simulink model "ADRC_PTAR2"  (R2025b)
settings: Solver=VariableStepAuto  StartTime=0.0  StopTime=500000  RelTol=1e-3
undefined symbols (not defined in the file): a0, a1, a2, a3, a4, a5, A_o, b0, Bau, denC, denGpi, E1, K, k, L, L_E, m, numC, numGpi, P_, Tau, Y_A, Y_H
libraries: slpidlib x1
settings Model: Creator=esteban  LastModifiedBy=esteban

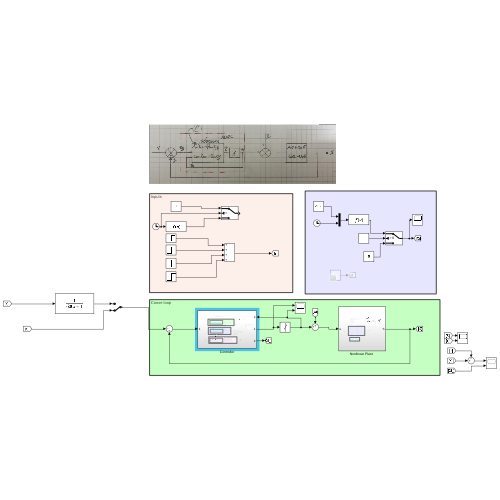
[thumbnail: Simulink's stored preview of the top-level diagram]
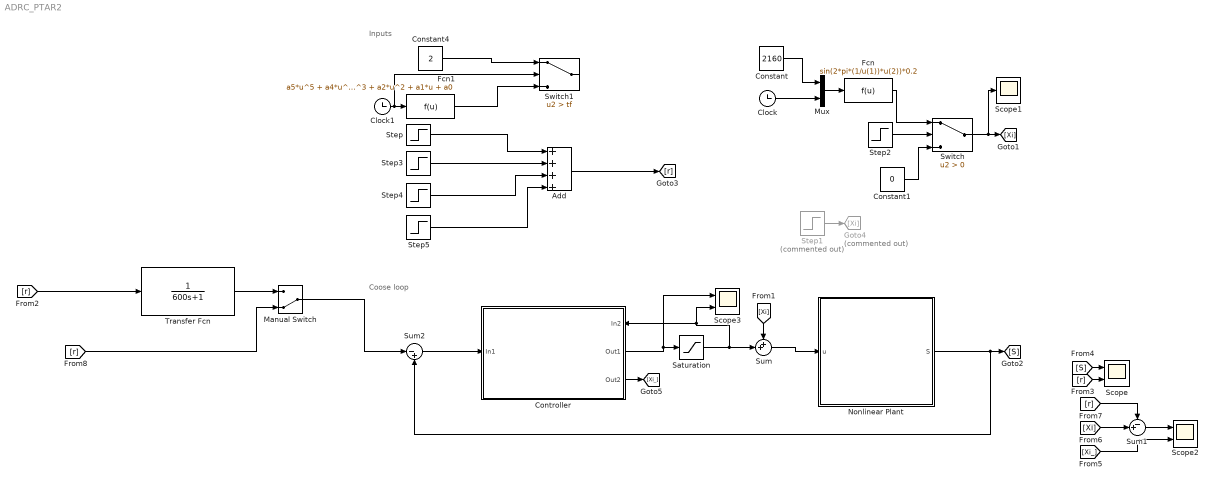
== system ADRC_PTAR2 ==
  note: Inputs
  note: Coose loop
  Add : Sum  Inputs=++++
  Clock : Clock
  Clock1 : Clock
  Constant : Constant  Value=2160
  Constant1 : Constant  Value=0
  Constant4 : Constant  Value=2
  Controller : Subsystem
      settings: PortSchema="{\"entries\":[{\"content\":{\"sides\":[{\"content\":{\"connectorIds\":[\"In1\"]},\"type\":\"ConnectorPlacement.EquallySpacedRectSide\",\"uuid\":\"f8461a81-2045-427e-a01f-edb502a076ed\"},{\"content\":{\"connectorIds\":[\"In2\",\"Out1\",\"Out2\"],\"side\":\"RIGHT\"},\"type\":\"ConnectorPlacement.EquallySpacedRectSide\",\"uuid\":\"3759dbef-32e7-4c7e-81ac-95d511493371\"},{\"content\":{\"side\":\"TOP\"},\"type\":\"ConnectorPlacement.EquallySpacedRectSide\",\"uuid\":\"15238c06-ddee-41c5-98cd-ddd7661e75a4\"}]},\"type\":\"ConnectorPlacement.EquallySpacedConnector\",\"uuid\":\"b42b1071-4ba9-4a20-bc2c-50f933ed0d4a\"}],\"packageUris\":[\"http://schema.mathworks.com/mf0/Connector/R2020b\"],\"version\":\"1.0\"}"
  Fcn : Fcn  Expr=sin(2*pi*(1/u(1))*u(2))*0.2
  Fcn1 : Fcn  Expr=a5*u^5 + a4*u^4 + a3*u^3 + a2*u^2 + a1*u + a0
  Goto4 : Goto  Commented=on  GotoTag=Xi
  Manual Switch : ManualSwitch  CurrentSetting=0
  Mux : Mux  Inputs=2
  "Nonlinear Plant  " : Subsystem
  Saturation : Saturate  UpperLimit=100  LowerLimit=0
  Scope : Scope  NumInputPorts=2
      settings: ActiveDisplayYMinimum=0.10311657808400376  ActiveDisplayYMaximum=3.8920516951737838
  Scope1 : Scope
      settings: ActiveDisplayYMinimum=-0.024830958943548569  ActiveDisplayYMaximum=0.2234786304919372  DataLoggingVariableName=ScopeData2
  Scope2 : Scope  NumInputPorts=2
      settings: ActiveDisplayYMinimum=-2.2923205992555511  ActiveDisplayYMaximum=4.2391627723615954  DataLoggingVariableName=ScopeData3
  Scope3 : Scope  NumInputPorts=2
      settings: ActiveDisplayYMinimum=-13.796251760586394  ActiveDisplayYMaximum=71.9907618847564  DataLoggingVariableName=ScopeData4
  Step : Step  Time=40000  After=2  SampleTime=0
  Step1 : Step  Commented=on  Time=4000  After=0.1  SampleTime=0
  Step2 : Step  Time=4000  SampleTime=0
  Step3 : Step  Time=80000  After=0.4  SampleTime=0
  Step4 : Step  Time=120000  After=-0.9  SampleTime=0
  Step5 : Step  Time=160000  After=0.5  SampleTime=0
  Sum : Sum  Inputs=++|
  Sum1 : Sum  Inputs=-+|
  Sum2 : Sum  Inputs=|-+
  Switch : Switch  Criteria=u2 > Threshold  SaturateOnIntegerOverflow=off  InputSameDT=off
  Switch1 : Switch  Criteria=u2 > Threshold  Threshold=tf  SaturateOnIntegerOverflow=off  InputSameDT=off
  Transfer Fcn : TransferFcn  Denominator=[600 1]
  wires:
  Mux/1 -> Fcn/1
  Clock/1 -> Mux/2
  Constant/1 -> Mux/1
  Step1/1 -> Goto4/1
  "Nonlinear Plant  "/1(S) -> [S], Sum2/2
  Constant1/1 -> Switch/3
  Fcn/1 -> Switch/1
  Step2/1 -> Switch/2
  Switch/1 -> Scope1/1, [Xi]
  [r] -> Scope/2
  Controller/2(Out2) -> [Xi_]
  [S] -> Scope/1
  [Xi_] -> Scope2/2
  Sum1/1 -> Scope2/1
  [r] -> Sum1/1
  Step/1 -> Add/1
  Step3/1 -> Add/2
  Step4/1 -> Add/3
  Step5/1 -> Add/4
  [Xi] -> Sum1/2
  Sum2/1 -> Controller/1(In1)
  [r] -> Transfer Fcn/1
  Manual Switch/1 -> Sum2/1
  Transfer Fcn/1 -> Manual Switch/1
  Sum/1 -> "Nonlinear Plant  "/1(u)
  Controller/1(Out1) -> Saturation/1, Scope3/1
  [r] -> Manual Switch/2
  Constant4/1 -> Switch1/1
  Clock1/1 -> Switch1/2, Fcn1/1
  Fcn1/1 -> Switch1/3
  Add/1 -> [r]
  Saturation/1 -> Scope3/2, Controller/2(In2), Sum/2
  [Xi] -> Sum/1

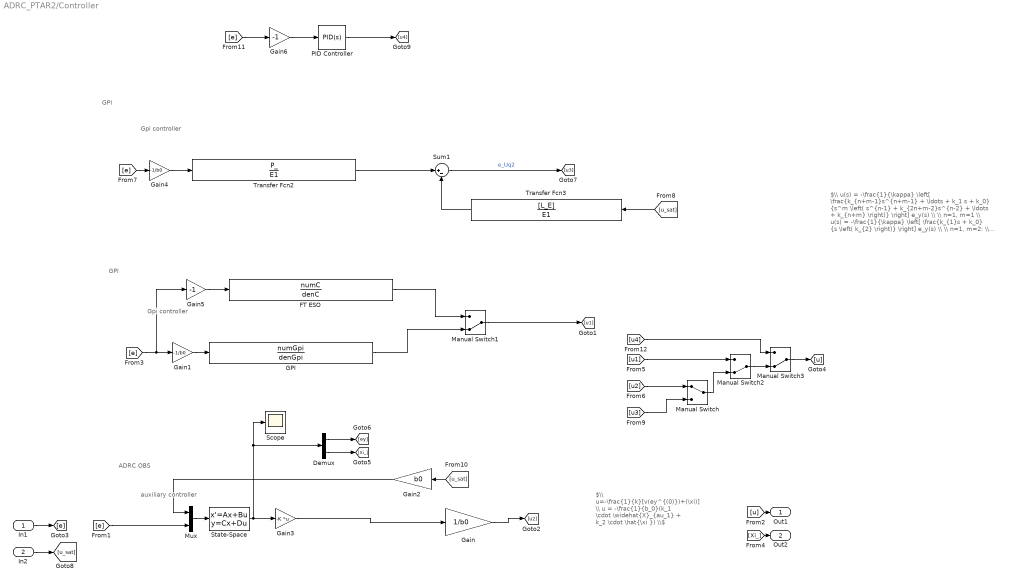
== system ADRC_PTAR2/Controller ==
  note: $\\ u(s) = -\frac{1}{\kappa} \left[ \frac{k_{n+m-1}s^{n+m-1} + \ldots + k_1 s + k_0} {s^m \left( s^{n-1} + k_{2n+m-2}s^{n-2} + \ldots + k_{n+m} \right)} \right] e_y(s) \\ \\ n=1, m=1 \\ u(s) = -\frac{1}{\kappa} \left[ \frac{k_{1}s + k_0} {s \left( k_{2} \right)} \right] e_y(s) \\ \\ n=1, m=2: \\ u(s) = -\frac{1}{b_0} \left[ \frac{k_{2}s^2+k_{1}s + k_0} {s^2} \right] e_y(s)$
  note: $\\ u=-\frac{1}{k}[v(ey^{(0)})+(\xi)] \\ u = -\frac{1}{b_0}(k_1 \cdot \widehat{X}_{au_1} + k_2 \cdot \hat{\xi }) \\$
  note: auxiliary controller
  note: Gpi controller
  note: GPI
  note: ADRC OBS
  note: GPI
  note: Gpi controller
  In1 : Inport
  In2 : Inport  Port=2
  Demux : Demux  Outputs=2
  FT ESO : TransferFcn  Numerator=numC  Denominator=denC
  GPI : TransferFcn  Numerator=numGpi  Denominator=denGpi
  Gain : Gain  Gain=1/b0
  Gain1 : Gain  Gain=-1/b0
  Gain2 : Gain  Gain=b0
  Gain3 : Gain  Gain=-K  Multiplication=Matrix(K*u)
  Gain4 : Gain  Gain=-1/b0
  Gain5 : Gain  Gain=-1
  Gain6 : Gain  Gain=-1
  Manual Switch : ManualSwitch
  Manual Switch1 : ManualSwitch  CurrentSetting=0
  Manual Switch2 : ManualSwitch  CurrentSetting=0
  Manual Switch3 : ManualSwitch  CurrentSetting=0
  Mux : Mux  Inputs=2
  PID Controller : slpidlib/PID Controller  Controller=PID  Form=Ideal  TimeDomain=Continuous-time  UseExternalTs=off  SampleTime=-1  IntegratorMethod=Forward Euler  FilterMethod=Forward Euler  ControllerParametersSource=internal  P=490.3  I=1/134.1  UseKiTs=off  D=14.78  UseExternalDerivativeSource=off  N=1/1.48  UseFilter=on  TunerSelectOption=Transfer Function Based (PID Tuner App)  InitialConditionSource=internal  InitialConditionForIntegrator=0  InitialConditionForFilter=0  DifferentiatorICPrevScaledInput=0  ExternalReset=none  TrackingMode=off  Kt=1  LimitOutput=off  SatLimitsSource=internal  UpperSaturationLimit=inf  LowerSaturationLimit=-inf  LinearizeAsGain=on  AntiWindupMode=none  Kb=1  LimitIntegrator=off  UpperIntegratorSaturationLimit=inf  LowerIntegratorSaturationLimit=-inf  POutMin=[]  POutMax=[]  IOutMin=[]  IOutMax=[]  DOutMin=[]  DOutMax=[]  NOutMin=[]  NOutMax=[]  SumOutMin=[]  SumOutMax=[]  SaturationOutMin=[]  SaturationOutMax=[]  PParamMin=[]  PParamMax=[]  IParamMin=[]  IParamMax=[]  DParamMin=[]  DParamMax=[]  NParamMin=[]  NParamMax=[]  KbParamMin=[]  KbParamMax=[]  KtParamMin=[]  KtParamMax=[]  KbOutMin=[]  KbOutMax=[]  KtOutMin=[]  KtOutMax=[]  IntegratorOutMin=[]  IntegratorOutMax=[]  FilterOutMin=[]  FilterOutMax=[]  SumI1OutMin=[]  SumI1OutMax=[]  SumI2OutMin=[]  SumI2OutMax=[]  SumI3OutMin=[]  SumI3OutMax=[]  SumI4OutMin=[]  SumI4OutMax=[]  SumDOutMin=[]  SumDOutMax=[]  DifferentiatorOutMin=[]  DifferentiatorOutMax=[]  FilterDiffOutCoefMin=[]  FilterDiffOutCoefMax=[]  ReciprocalOutMin=[]  ReciprocalOutMax=[]  SumDenOutMin=[]  SumDenOutMax=[]  SumNumOutMin=[]  SumNumOutMax=[]  DivideOutMin=[]  DivideOutMax=[]  UdiffTsProdOutMin=[]  UdiffTsProdOutMax=[]  NTsProdOutMin=[]  NTsProdOutMax=[]  UintegralTsProdOutMin=[]  UintegralTsProdOutMax=[]  UngainTsProdOutMin=[]  UngainTsProdOutMax=[]  ClampingZeroOutDataTypeStr=Inherit: Inherit via back propagation  ClampingZeroOutMin=[]  ClampingZeroOutMax=[]  FilterDenConstantOutDataTypeStr=Inherit: Inherit via back propagation  FilterDenConstantOutMin=[]  FilterDenConstantOutMax=[]  PCopyOutDataTypeStr=Inherit: Inherit via back propagation  PCopyOutMin=[]  PCopyOutMax=[]  NCopyOutDataTypeStr=Inherit: Inherit via back propagation  NCopyOutMin=[]  NCopyOutMax=[]  IntegratorContinuousStateAttributes=''  IntegratorStateMustResolveToSignalObject=off  IntegratorRTWStateStorageClass=Auto  FilterContinuousStateAttributes=''  FilterStateMustResolveToSignalObject=off  FilterRTWStateStorageClass=Auto  ParallelPVariant=Passthrough  IdealPVariant=InternalParameters  IVariant=InternalParameters  DVariant=InternalParameters  IntegratorVariant=Continuous  SatVariant=Disabled  AWVariant=Passthrough  PCopyVariant=Disabled  TRVariant=Disabled  FdbkBlocksVariant=Forward  IdealPFdbkVariant=Disabled  SatFdbkVariant=Disabled  DerivativeFilterVariant=ContFilter  NVariant=InternalParameters  NCopyVariant=Disabled  FilterICVariant=InternalICsFilter  IntegratorICVariant=InternalICs  ExternalResetVariant=Disabled  TRSumVariant=Passthrough  SumFdbkVariant=Disabled  SumVariant=Sum_PID  TsampFilterVariant=InternalTs  TsampNgainVariant=Passthrough  TsampIntegralVariant=Disabled_SignalSpec  ExternalSaturationOutDataTypeStr=Inherit: Same as second input  DerivativeSourceVariant=ErrorSignal  PreIntVariant=InternalPreInt
  Scope : Scope
      settings: ActiveDisplayYMinimum=-0.028041843832660458  ActiveDisplayYMaximum=0.046633908399780717
  State-Space : StateSpace  A=A_o  B=[Bau L]  C=eye(m)  D=zeros(m,2)  InitialCondition=0
  Sum1 : Sum  Inputs=|+-
  Transfer Fcn2 : TransferFcn  Numerator=P_  Denominator=E1
  Transfer Fcn3 : TransferFcn  Numerator=[L_E]  Denominator=E1
  Out1 : Outport
  Out2 : Outport  Port=2
  wires:
  Mux/1 -> State-Space/1
  Gain3/1 -> Gain/1
  In1/1 -> [e]
  [u] -> Out1/1
  State-Space/1 -> Scope/1, Demux/1, Gain3/1
  Demux/2 -> [Xi_]
  Demux/1 -> [ey]
  [Xi_] -> Out2/1
  Gain/1 -> [u2]
  [e] -> Gain4/1
  Transfer Fcn3/1 -> Sum1/2
  In2/1 -> [u_sat]
  Sum1/1 -> [u3]  "e_Uq2"
  Transfer Fcn2/1 -> Sum1/1
  GPI/1 -> Manual Switch1/2
  FT ESO/1 -> Manual Switch1/1
  Manual Switch1/1 -> [u1]
  Manual Switch/1 -> Manual Switch2/2
  [u1] -> Manual Switch2/1
  [u2] -> Manual Switch/1
  [u3] -> Manual Switch/2
  [u_sat] -> Gain2/1
  Gain2/1 -> Mux/1
  [u_sat] -> Transfer Fcn3/1
  [e] -> Mux/2
  [e] -> Gain1/1, Gain5/1
  Gain4/1 -> Transfer Fcn2/1
  Gain5/1 -> FT ESO/1
  Gain1/1 -> GPI/1
  [e] -> Gain6/1
  Gain6/1 -> PID Controller/1
  Manual Switch2/1 -> Manual Switch3/2
  Manual Switch3/1 -> [u]
  PID Controller/1 -> [u4]
  [u4] -> Manual Switch3/1

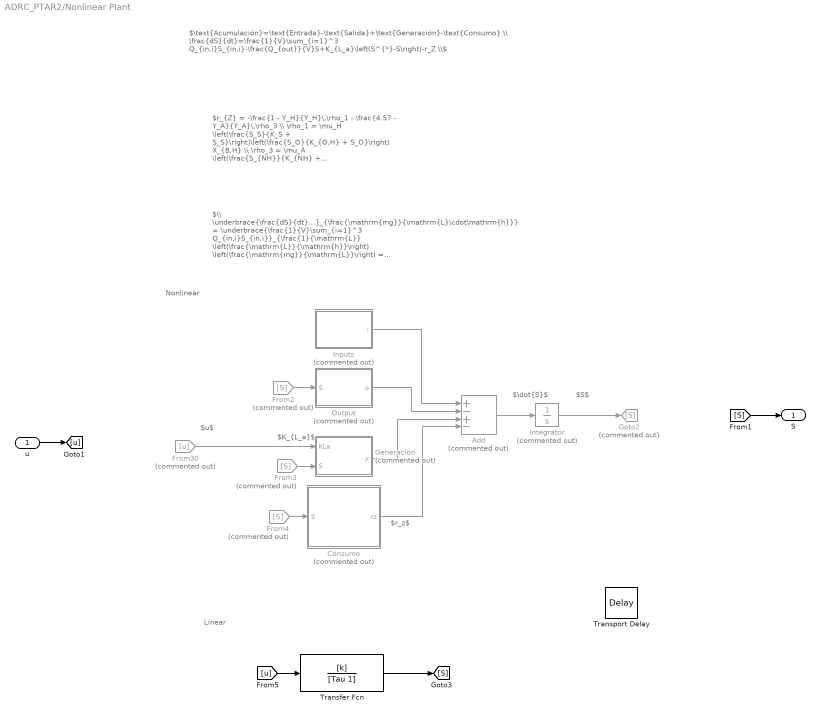
== system ADRC_PTAR2/Nonlinear Plant   ==
  note: Linear
  note: Nonlinear
  note: $\dot{S}$
  note: $\\ \underbrace{\frac{dS}{dt}}_{\frac{\mathrm{mg}}{\mathrm{L}\cdot\mathrm{h}}} = \underbrace{\frac{1}{V}\sum_{i=1}^3 Q_{in,i}S_{in,i}}_{\frac{1}{\mathrm{L}} \left(\frac{\mathrm{L}}{\mathrm{h}}\right) \left(\frac{\mathrm{mg}}{\mathrm{L}}\right) = \frac{\mathrm{mg}}{\mathrm{L}\cdot\mathrm{h}}} - \underbrace{\frac{Q_{out}}{V}S}_{\left(\frac{\mathrm{L}/\mathrm{h}}{\mathrm{L}}\right) \left(\frac{\mathrm{mg}}{\mathrm{L}}\right) = \frac{\mathrm{mg}}{\mathrm{L}\cdot\mathrm{h}}} + \underbrace{K_{La}(S^{*}-S)}_{\left(\frac{1}{\mathrm{h}}\right) \left(\frac{\mathrm{mg}}{\mathrm{L}}\right) = \frac{\mathrm{mg}}{\mathrm{L}\cdot\mathrm{h}}} - \underbrace{r_Z}_{\frac{\mathrm{mg}}{\mathrm{L}\cdot\mathrm{h}}}$
  note: $r_{Z} = -\frac{1 - Y_H}{Y_H}\,\rho_1 - \frac{4.57 - Y_A}{Y_A}\,\rho_3 \\ \rho_1 = \mu_H \left(\frac{S_S}{K_S + S_S}\right)\left(\frac{S_O}{K_{O,H} + S_O}\right) X_{B,H} \\ \rho_3 = \mu_A \left(\frac{S_{NH}}{K_{NH} + S_{NH}}\right)\left(\frac{S_O}{K_{O,A} + S_O}\right) X_{B,A}$
  note: $\text{Acumulación}=\text{Entrada}-\text{Salida}+\text{Generación}-\text{Consumo} \\ \frac{dS}{dt}=\frac{1}{V}\sum_{i=1}^3 Q_{in,i}S_{in,i}-\frac{Q_{out}}{V}S+K_{L_a}\left(S^{*}-S\right)-r_Z \\$
  note: $S$
  note: $u$
  note: $K_{L_a}$
  note: $r_z$
  u : Inport
  Add : Sum  Commented=on  Inputs=+-+-
  Consumo : Subsystem  Commented=on
  From2 : From  Commented=on  GotoTag=S
  From3 : From  Commented=on  GotoTag=S
  From30 : From  Commented=on  GotoTag=u
  From4 : From  Commented=on  GotoTag=S
  Generacion : MATLAB Function  Commented=on  TreatAsAtomicUnit=on
  Goto2 : Goto  Commented=on  GotoTag=S
  Inputs : MATLAB Function  Commented=on  TreatAsAtomicUnit=on
  Integrator : Integrator  Commented=on
  Output : MATLAB Function  Commented=on  TreatAsAtomicUnit=on
  Transfer Fcn : TransferFcn  Numerator=[k]  Denominator=[Tau 1]
  Transport Delay : TransportDelay  DelayTime=50
  S : Outport
  wires:
  Add/1 -> Integrator/1
  From30/1 -> Generacion/1(KLa)
  Consumo/1(rz) -> Add/4
  Generacion/1(y) -> Add/3
  Output/1(o) -> Add/2
  Inputs/1(i) -> Add/1
  Integrator/1 -> Goto2/1
  u/1 -> [u]
  [S] -> S/1
  From2/1 -> Output/1(S)
  From3/1 -> Generacion/2(S)
  From4/1 -> Consumo/1(S)
  Transfer Fcn/1 -> [S]
  [u] -> Transfer Fcn/1

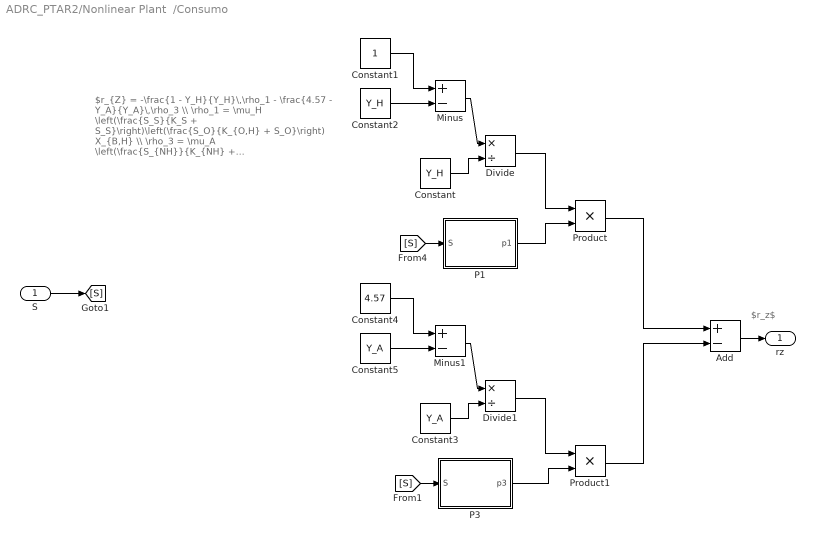
== system ADRC_PTAR2/Nonlinear Plant  /Consumo ==
  note: $r_z$
  note: $r_{Z} = -\frac{1 - Y_H}{Y_H}\,\rho_1 - \frac{4.57 - Y_A}{Y_A}\,\rho_3 \\ \rho_1 = \mu_H \left(\frac{S_S}{K_S + S_S}\right)\left(\frac{S_O}{K_{O,H} + S_O}\right) X_{B,H} \\ \rho_3 = \mu_A \left(\frac{S_{NH}}{K_{NH} + S_{NH}}\right)\left(\frac{S_O}{K_{O,A} + S_O}\right) X_{B,A}$
  S : Inport
  Add : Sum  Inputs=+-
  Constant : Constant  Value=Y_H
  Constant1 : Constant
  Constant2 : Constant  Value=Y_H
  Constant3 : Constant  Value=Y_A
  Constant4 : Constant  Value=4.57
  Constant5 : Constant  Value=Y_A
  Divide : Product  Inputs=*/
  Divide1 : Product  Inputs=*/
  Minus : Sum  Inputs=+-
  Minus1 : Sum  Inputs=+-
  P1 : MATLAB Function  TreatAsAtomicUnit=on
  P3 : MATLAB Function  TreatAsAtomicUnit=on
  Product : Product
  Product1 : Product
  rz : Outport
  wires:
  Add/1 -> rz/1
  P1/1(p1) -> Product/2
  Divide/1 -> Product/1
  Constant/1 -> Divide/2
  Constant2/1 -> Minus/2
  Constant1/1 -> Minus/1
  Minus/1 -> Divide/1
  Product/1 -> Add/1
  Minus1/1 -> Divide1/1
  P3/1(p3) -> Product1/2
  Constant3/1 -> Divide1/2
  Divide1/1 -> Product1/1
  Constant5/1 -> Minus1/2
  Constant4/1 -> Minus1/1
  Product1/1 -> Add/2
  S/1 -> [S]
  [S] -> P1/1(S)
  [S] -> P3/1(S)

== matlab function ADRC_PTAR2/Nonlinear Plant  /Inputs ==
  data: i output
function i = fcn()
coder.extrinsic('evalin',"assignin");
Q_1 = zeros(1,1);
Q_1 = double(evalin('base', 'Q_1'));
Q_2 = zeros(1,1);
Q_2 = double(evalin('base', 'Q_2'));
Q_3 = zeros(1,1);
Q_3 = double(evalin('base', 'Q_3'));

S_1 = zeros(1,1);
S_1 = double(evalin('base', 'S_1'));
S_2 = zeros(1,1);
S_2 = double(evalin('base', 'S_2'));
S_3 = zeros(1,1);
S_3 = double(evalin('base', 'S_3'));

V = zeros(1,1);
V = double(evalin('base', 'V'));

i = (Q_1*S_O1+Q_2*S_O2+Q_3*S_O3)/V;

== matlab function ADRC_PTAR2/Nonlinear Plant  /Output ==
  data: o output; S input
function o = fcn(S)
coder.extrinsic('evalin',"assignin");
Q_out = zeros(1,1);
Q_out = double(evalin('base', 'Q_out'));
V = zeros(1,1);
V = double(evalin('base', 'V'));
o = (Q_out/V)*S;

== matlab function ADRC_PTAR2/Nonlinear Plant  /Generacion ==
  data: KLa input; y output; S input
function y = fcn(KLa,S)
coder.extrinsic('evalin',"assignin");
S_O_SAT = zeros(1,1);
S_O_SAT = double(evalin('base', 'S_O_SAT'));
y =KLa (S_O_SAT-S);

== matlab function ADRC_PTAR2/Nonlinear Plant  /Consumo/P1 ==
  data: p1 output; S input
function p1 = fcn(S)
coder.extrinsic('evalin',"assignin");
mu_H = zeros(1,1);
mu_H = double(evalin('base', 'mu_H'));
S_S = zeros(1,1);
S_S = double(evalin('base', 'S_S'));
K_S = zeros(1,1);
K_S = double(evalin('base', 'K_S'));
K_OH = zeros(1,1);
K_OH = double(evalin('base', 'K_OH'));
X_BH = zeros(1,1);
X_BH = double(evalin('base', 'X_BH'));
p1 = mu_H*(S_S/(K_S+S_S))*(S/(K_OH+S))*X_BH;

== matlab function ADRC_PTAR2/Nonlinear Plant  /Consumo/P3 ==
  data: p3 output; S input
function p3 = fcn(S)
coder.extrinsic('evalin',"assignin");
mu_A = zeros(1,1);
mu_A = double(evalin('base', 'mu_A'));
S_NH = zeros(1,1);
S_NH = double(evalin('base', 'S_NH'));
K_NH = zeros(1,1);
K_NH = double(evalin('base', 'K_NH'));
K_OA = zeros(1,1);
K_OA = double(evalin('base', 'K_OA'));
X_BA = zeros(1,1);
X_BA = double(evalin('base', 'X_BA'));
p3 = mu_A*(S_NH/(K_NH+S_NH))*(S/(K_OA+S))*X_BA;
